simulink model "TemperatureControl_Minima"  (R2026a)
settings: Solver=FixedStepAuto  StopTime=inf  FixedStep=0.1  EnableMultiTasking=on
libraries: arduinolib x6
settings Model: SILPILModeSetting=veronly  ExtModeTrigDuration=2  Creator=arkad  LastModifiedBy=arkad
settings HardwareCC: ProdLargestAtomicInteger=Long  ProdLargestAtomicFloat=Double  ProdHWDeviceType=ARM Compatible->ARM Cortex
settings RTWCC: SystemTargetFile=ert.tlc  HardwareBoard=Arduino Uno R4 Minima  TLCOptions=-aInlineSetEventsForThisBaseRateFcn=TLC_FALSE -aSuppressMultiTaskScheduler=TLC_FALSE -aRateBasedStepFcn=1  Toolchain=Arduino ARM M4  BuildConfiguration=Faster Runs  Description=Embedded Coder
settings ERTTargetCC: ExtModeTransport=3.0  ExtModeAutomaticAllocSize=off  ExtModeStaticAllocSize=8192.0  SupportContinuousTime=on  SupportVariableSizeSignals=on

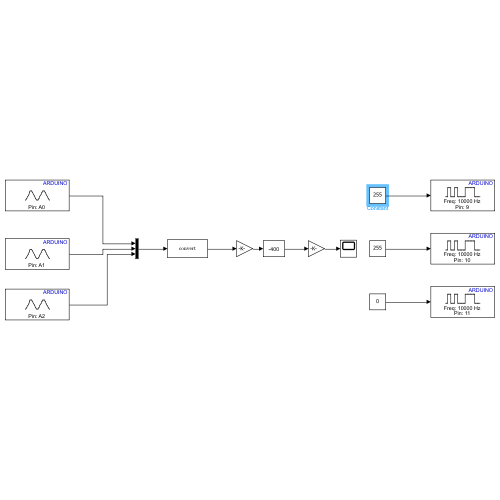
[thumbnail: Simulink's stored preview of the top-level diagram]
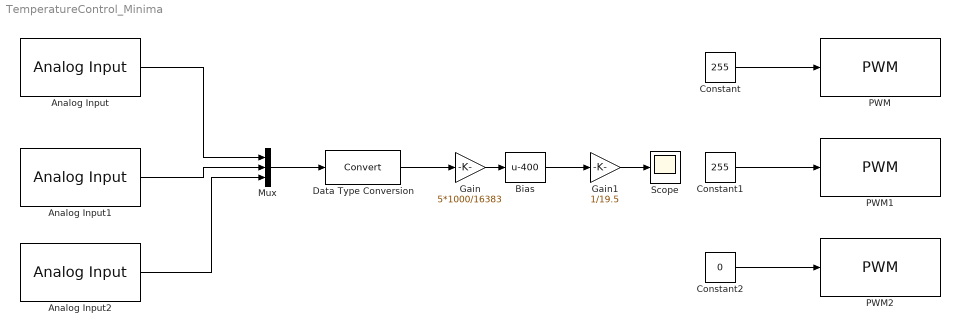
== system TemperatureControl_Minima ==
  Analog Input : arduinolib/Analog Input  pinNumber=0  ReadResultsOnly=off  ConversionTriggerSource=Software  ExternalTriggerType=uint32( 0 )  OutputDataType=uint16  EnableConversionCompleteNotify=off  EnableOuputStatus=off  SampleTime=-1  blockPlatform=arduino
  Analog Input1 : arduinolib/Analog Input  pinNumber=1  ReadResultsOnly=off  ConversionTriggerSource=Software  ExternalTriggerType=uint32( 0 )  OutputDataType=uint16  EnableConversionCompleteNotify=off  EnableOuputStatus=off  SampleTime=-1  blockPlatform=arduino
  Analog Input2 : arduinolib/Analog Input  pinNumber=2  ReadResultsOnly=off  ConversionTriggerSource=Software  ExternalTriggerType=uint32( 0 )  OutputDataType=uint16  EnableConversionCompleteNotify=off  EnableOuputStatus=off  SampleTime=-1  blockPlatform=arduino
  Bias : Bias  Bias=-400  SaturateOnIntegerOverflow=off
  Constant : Constant  Value=255
  Constant1 : Constant  Value=255
  Constant2 : Constant  Value=0
  Data Type Conversion : DataTypeConversion  SaturateOnIntegerOverflow=off  RndMeth=Floor
  Gain : Gain  Gain=5*1000/16383
  Gain1 : Gain  Gain=1/19.5
  Mux : Mux  Inputs=3
  PWM : arduinolib/PWM  pinNumber=9  frequencyType=Specify  desiredFrequency=10000  achievableFrequency=10000
  PWM1 : arduinolib/PWM  pinNumber=10  frequencyType=Specify  desiredFrequency=10000  achievableFrequency=10000
  PWM2 : arduinolib/PWM  pinNumber=11  frequencyType=Specify  desiredFrequency=10000  achievableFrequency=10000
  Scope : Scope
      settings: TimeSpan=100  ActiveDisplayYMinimum=25  ActiveDisplayYMaximum=125
  wires:
  Constant/1 -> PWM/1
  Analog Input1/1 -> Mux/2
  Analog Input2/1 -> Mux/3
  Analog Input/1 -> Mux/1
  Mux/1 -> Data Type Conversion/1
  Gain1/1 -> Scope/1
  Gain/1 -> Bias/1
  Bias/1 -> Gain1/1
  Data Type Conversion/1 -> Gain/1
  Constant1/1 -> PWM1/1
  Constant2/1 -> PWM2/1
